simulink model "forty_gbe"  (R2019a)
settings: Solver=VariableStepAuto  StartTime=0.0  StopTime=10.0  RelTol=1e-3
libraries: xbsIndex_r4 x1231, casper_library_misc x9
(part 5 of 14)

== system forty_gbe/forty_gbe/rxs2/arm_delay ==
  d : Inport
  q : Outport
  wires:
  d/1 -> q/1

== system forty_gbe/forty_gbe/rxs2/buscreate ==
  in1 : Inport
  reinterpret1 : xbsIndex_r4/Reinterpret  force_arith_type=on  arith_type=Unsigned  force_bin_pt=on  bin_pt=0  block_type=reinterpret
      settings: infoedit="Changes signal type without altering the binary representation.   You can changed the signal between signed and unsigned, and relocate the binary point.<br><br>Hardware notes: In hardware this block costs nothing.<br><br>Example:  Suppose the input is 6 bits wide, signed, with 2 fractional bits, and the output is forced to unsigned with 0 fractional bits.  Then an input of -2.0 (1110.00 in binary 2's complement) becomes an output of 56 (111000 in binary)."
  bus_out : Outport
  wires:
  in1/1 -> reinterpret1/1
  reinterpret1/1 -> bus_out/1

== system forty_gbe/forty_gbe/rxs2/io_delay ==
  d : Inport
  Register0 : xbsIndex_r4/Register  init=0  rst=off  en=off  dbl_ovrd=off  block_type=register
      settings: block_version=11.4
  Register1 : xbsIndex_r4/Register  init=0  rst=off  en=off  dbl_ovrd=off  block_type=register
      settings: block_version=11.4
  q : Outport
  wires:
  Register1/1 -> q/1
  d/1 -> Register0/1
  Register0/1 -> Register1/1

== system forty_gbe/forty_gbe/rxs2/ss ==
  note: Generate stop
      | when in circular
      | capture mode
  note: Delay start
      | of capture
  note: ctrl:
      | bit0: Put a posedge here
      |         to enable a new capture.
      | bit1: ignore external trigger
      |         and trigger immediately.
      | bit2: ignore external write
      |         enable and capture on
      |         every FPGA clock.
      | bit3: continuously capture
      |         data until we get an
      |         external stop command.
  note: Offset in vector
      | from first element
      | captured, used
      | during circular capture
  note: Number of
      | bytes in
      | buffer and
      | done bit
  note: Number of valid
      | data samples to
      | skip after trigger
      | before starting
      | capture
  note: Value on vin
      | aligned with
      | first sample on
      | din captured
  din : Inport
  we : Inport  Port=2
  trig : Inport  Port=3
  arm : Inport  Port=4
  add_del : xbsIndex_r4/Delay  rst=off  infoeditControl=Selection of Reset will increase slice count due to use of real FFs and instead of SRLs  en=off  latency=1  reg_retiming=on  dbl_ovrd=off  block_type=delay
      settings: block_version=11.4
  add_gen : Subsystem  AncestorBlock=casper_library_scopes/snapshot/add_gen  mask{counter_size=10+4+1, increment=16, nsamples=10, burst_size=0, use_dsp48=on}
      mask prompts: counter_size "Address counter size (2^?)"; increment "Address counter increment"; nsamples "Number of samples (2^?)"; burst_size "Burst size (2^?)"; use_dsp48 "dsp48 counter/s"
      mask init:
      | set_param(gcb,'LinkStatus','inactive');
      | if strcmp(use_dsp48,'on'),
      |     set_param([gcb,'/add_gen'],'implementation','DSP48');
      | else
      |     set_param([gcb,'/add_gen'],'implementation','Fabric');
      | end
  arm_or : xbsIndex_r4/Logical  logical_function=OR  inputs=2  en=off  latency=0  precision=Full  arith_type=Unsigned  n_bits=16  bin_pt=0  align_bp=on  dbl_ovrd=off  block_type=logical
  basic_ctrl : Subsystem  AncestorBlock=casper_library_scopes/snapshot/basic_ctrl  mask{dram=off, data_width=128}
      mask prompts: data_width "data width"
      mask init:
      | set_param(gcb,'LinkStatus','inactive');
      | set_param([gcb,'/dram_munge'], 'dram', dram);
  bram : Subsystem  Tag=xps:bram  AncestorBlock=xps_library/Memory/shared_bram  mask{arith_type=Unsigned, addr_width=10, data_width=128, reg_prim_output=off, reg_core_output=off, optimization=Minimum_Area, data_bin_pt=0, init_vals=[0:2^10-1], sample_rate=1}
      mask prompts: arith_type "Output Data Type"; addr_width "Address width"; data_width "Data Width"; reg_prim_output "Register Primitive Output"; reg_core_output "Register Core Output"; data_bin_pt "Data Binary Point"; init_vals "Initial values (simulation only)"; sample_rate "Sample rate"
      mask init:
      | shared_bram_mask;
      mask TypeOptions arith_type: Unsigned | Signed  (2's comp)
      mask TypeOptions data_width: 8 | 16 | 32 | 64 | 128
      mask TypeOptions optimization: Minimum_Area | Low_Power
  cast : xbsIndex_r4/Convert  gui_display_data_type=Fixed-point  arith_type=Unsigned  n_bits=128  bin_pt=0  float_type=Single  exp_bits=8  fraction_bits=24  quantization=Truncate  overflow=Wrap  en=off  latency=0  pipeline=off  dbl_ovrd=off  block_type=convert
      settings: block_version=11.4
  circ : xbsIndex_r4/Constant  const=0  gui_display_data_type=Fixed-point  arith_type=Boolean  n_bits=16  bin_pt=14  preci_type=Single  exp_width=8  frac_width=24  explicit_period=on  period=1  equ=P=C  opselect=C  inp2=PCIN>>17  opr=+  inp1=P  carry=CIN  dbl_ovrd=off  block_type=constant
  circ_or : xbsIndex_r4/Logical  logical_function=OR  inputs=2  en=off  latency=0  precision=Full  arith_type=Unsigned  n_bits=16  bin_pt=0  align_bp=on  dbl_ovrd=off  block_type=logical
  ctrl : Subsystem  Tag=xps:sw_reg  AncestorBlock=xps_library/Memory/software_register  mask(swreg){io_dir=From Processor, io_delay=0, init_val=0, sample_period=1, names=reg, bitwidths=32, bin_pts=0, arith_types=0, sim_port=off, show_format=on}
      mask prompts: io_dir "I/O direction"; io_delay "I/O delay"; init_val "Initial Value"; sample_period "Sample period"; names "Bitfield names [msb...lsb]"; bitwidths "Bitfield widths"; bin_pts "Bitfield binary pts"; arith_types "Bitfield types, ufix=0, fix=1, bool=2"; sim_port "Provide sim input/output?"; show_format "Print format string?"
      mask help: A 32-bit software-accessible register. Can be divided into bitfields of varying widths and types using the fields in the block mask.
      mask init:
      | swreg_init(gcb)
      settings: AttributesFormatString=1input:uf32.0 = 32 bits
      mask TypeOptions io_dir: To Processor | From Processor
      mask Callback io_dir:
      | mask_enables = get_param(gcb, 'MaskEnables');
      | mask_names = get_param(gcb, 'MaskNames');
      | if strcmp(get_param(gcb, 'io_dir'), 'To Processor'),
      |     mask_enables{ismember(mask_names, 'sample_period')} = 'off';
      | else
      |     mask_enables{ismember(mask_names, 'sample_period')} = 'on';
      | end
      | set_param(gcb, 'MaskEnables', mask_enables);
      mask DialogControl ParameterTabVar0 Prompt: Setup
  ctrl_combine : Subsystem  AncestorBlock=casper_library_flow_control/bus_create  mask(bus_create){inputNum=4}
      mask prompts: inputNum "Number of inputs:"
      mask init:
      | bus_create_init(gcb,...
      |     'inputNum', inputNum);
  ctrl_split : Subsystem  AncestorBlock=casper_library_flow_control/bus_expand  mask(bus_expand){mode=divisions of arbitrary size, outputNum=1, outputWidth=[28 1 2 1], outputBinaryPt=0, outputArithmeticType=[0 2 0 2], show_format=on, outputToWorkspace=off, variablePrefix=out, outputToModelAsWell=on}
      mask prompts: outputNum "Number of outputs:"; outputWidth "Output width [msb ... lsb]:"; outputBinaryPt "Output binary point position [msb ... lsb]:"; outputArithmeticType "Output arithmetic type (ufix=0, fix=1, bool=2) [msb ... lsb]:"; show_format "Print format string?"; outputToWorkspace "Output to workspace?"; variablePrefix "Variable name prefix:"; outputToModelAsWell "Output to model as well?"
      mask help:
      | Expands a 'bus' made using a bus_create or Xilinx
      | concat block.
      | The input will be divided into the specified number
      | of outputs with the specified arithmetic types.
      | Divisions are made from most significant bit.
      mask init: same as forty_gbe/forty_gbe/rx_dv_or_exp
      settings: AttributesFormatString=4 outputs: uf28.0,b,uf2.0,b,
      mask TypeOptions mode: divisions of equal size | divisions of arbitrary size
      mask Callback mode: bus_expand_callback();
      mask Callback outputWidth: bus_expand_callback();
      mask Callback outputToWorkspace: bus_expand_callback();
  dat_del : xbsIndex_r4/Delay  rst=off  infoeditControl=Selection of Reset will increase slice count due to use of real FFs and instead of SRLs  en=off  latency=1  reg_retiming=on  dbl_ovrd=off  block_type=delay
      settings: block_version=11.4
  g_tr_en_cnt : Terminator
  gbram : Terminator
  goto_ss_we2_const : xbsIndex_r4/Constant  const=0  gui_display_data_type=Fixed-point  arith_type=Boolean  n_bits=16  bin_pt=14  preci_type=Single  exp_width=8  frac_width=24  explicit_period=on  period=1  equ=P=C  opselect=C  inp2=PCIN>>17  opr=+  inp1=P  carry=CIN  dbl_ovrd=off  block_type=constant
  goto_ss_we3_const : xbsIndex_r4/Constant  const=0  gui_display_data_type=Fixed-point  arith_type=Boolean  n_bits=16  bin_pt=14  preci_type=Single  exp_width=8  frac_width=24  explicit_period=on  period=1  equ=P=C  opselect=C  inp2=PCIN>>17  opr=+  inp1=P  carry=CIN  dbl_ovrd=off  block_type=constant
  gval : Terminator
  never : xbsIndex_r4/Constant  const=0  gui_display_data_type=Fixed-point  arith_type=Boolean  n_bits=16  bin_pt=14  preci_type=Single  exp_width=8  frac_width=24  explicit_period=on  period=1  equ=P=C  opselect=C  inp2=PCIN>>17  opr=+  inp1=P  carry=CIN  dbl_ovrd=off  block_type=constant
  ri : xbsIndex_r4/Reinterpret  force_arith_type=on  arith_type=Unsigned  force_bin_pt=on  bin_pt=0  block_type=reinterpret
      settings: infoedit="Changes signal type without altering the binary representation.   You can changed the signal between signed and unsigned, and relocate the binary point.<br><br>Hardware notes: In hardware this block costs nothing.<br><br>Example:  Suppose the input is 6 bits wide, signed, with 2 fractional bits, and the output is forced to unsigned with 0 fractional bits.  Then an input of -2.0 (1110.00 in binary 2's complement) becomes an output of 56 (111000 in binary)."
  status : Subsystem  Tag=xps:sw_reg  AncestorBlock=xps_library/Memory/software_register  mask(swreg){io_dir=To Processor, io_delay=0, init_val=0, sample_period=1, names=reg, bitwidths=32, bin_pts=0, arith_types=0, sim_port=off, show_format=on}
      mask prompts: io_dir "I/O direction"; io_delay "I/O delay"; init_val "Initial Value"; sample_period "Sample period"; names "Bitfield names [msb...lsb]"; bitwidths "Bitfield widths"; bin_pts "Bitfield binary pts"; arith_types "Bitfield types, ufix=0, fix=1, bool=2"; sim_port "Provide sim input/output?"; show_format "Print format string?"
      mask help: A 32-bit software-accessible register. Can be divided into bitfields of varying widths and types using the fields in the block mask.
      mask init:
      | swreg_init(gcb)
      settings: AttributesFormatString=1output:uf32.0 = 32 bits
      mask TypeOptions io_dir: To Processor | From Processor
      mask Callback io_dir:
      | mask_enables = get_param(gcb, 'MaskEnables');
      | mask_names = get_param(gcb, 'MaskNames');
      | if strcmp(get_param(gcb, 'io_dir'), 'To Processor'),
      |     mask_enables{ismember(mask_names, 'sample_period')} = 'off';
      | else
      |     mask_enables{ismember(mask_names, 'sample_period')} = 'on';
      | end
      | set_param(gcb, 'MaskEnables', mask_enables);
      mask DialogControl ParameterTabVar0 Prompt: Setup
  vin_const : xbsIndex_r4/Constant  const=0  gui_display_data_type=Fixed-point  arith_type=Boolean  n_bits=16  bin_pt=14  preci_type=Single  exp_width=8  frac_width=24  explicit_period=on  period=1  equ=P=C  opselect=C  inp2=PCIN>>17  opr=+  inp1=P  carry=CIN  dbl_ovrd=off  block_type=constant
  we_del : xbsIndex_r4/Delay  rst=off  infoeditControl=Selection of Reset will increase slice count due to use of real FFs and instead of SRLs  en=off  latency=1  reg_retiming=on  dbl_ovrd=off  block_type=delay
      settings: block_version=11.4
  arm_out : Outport
  tag scope: goto_51569036_we1=global, goto_51569036_we2=global, goto_51569036_we3=global, goto_51569036_we4=global
  wires:
  din/1 -> ri/1
  ri/1 -> cast/1
  cast/1 -> basic_ctrl/2(din)
  we/1 -> basic_ctrl/3(we)
  trig/1 -> basic_ctrl/4(trig)
  ctrl_combine/1(bus_out) -> basic_ctrl/5(ctrl)
  never/1 -> basic_ctrl/6(stopi)
  arm/1 -> arm_or/2
  arm_or/1 -> arm_out/1, ctrl_combine/4(in4)
  circ/1 -> circ_or/2
  ctrl/1(in_reg) -> ctrl_split/1(bus_in)
  ctrl_split/1(msb_out4) -> ctrl_combine/1(in1)
  ctrl_split/2(out3) -> circ_or/1
  ctrl_split/3(out2) -> ctrl_combine/3(in3)
  ctrl_split/4(lsb_out1) -> arm_or/1
  circ_or/1 -> ctrl_combine/2(in2)
  basic_ctrl/1(vout) -> add_gen/1(vin)
  basic_ctrl/2(dout) -> add_gen/2(din)
  basic_ctrl/3(we_o) -> add_gen/3(we), [goto_51569036_we1]
  basic_ctrl/4(go) -> add_gen/4(go)
  basic_ctrl/5(stop) -> add_gen/5(cont)
  basic_ctrl/6(init) -> add_gen/6(init)
  add_gen/5(status) -> status/1(out_reg)
  vin_const/1 -> basic_ctrl/1(vin)
  add_gen/1(vout) -> gval/1
  add_gen/6(en_cnt) -> g_tr_en_cnt/1
  add_gen/2(add) -> add_del/1
  add_gen/3(dout) -> dat_del/1
  add_gen/4(we_o) -> we_del/1, [goto_51569036_we4]
  add_del/1 -> bram/1(addr)
  dat_del/1 -> bram/2(data_in)
  we_del/1 -> bram/3(we)
  bram/1(data_out) -> gbram/1
  goto_ss_we2_const/1 -> [goto_51569036_we2]
  goto_ss_we3_const/1 -> [goto_51569036_we3]

== system forty_gbe/forty_gbe/rxs2/trig_delay ==
  d : Inport
  Register0 : xbsIndex_r4/Register  init=0  rst=off  en=off  dbl_ovrd=off  block_type=register
      settings: block_version=11.4
  Register1 : xbsIndex_r4/Register  init=0  rst=off  en=off  dbl_ovrd=off  block_type=register
      settings: block_version=11.4
  q : Outport
  wires:
  Register1/1 -> q/1
  d/1 -> Register0/1
  Register0/1 -> Register1/1

== system forty_gbe/forty_gbe/rxs2/we_delay ==
  d : Inport
  Register0 : xbsIndex_r4/Register  init=0  rst=off  en=off  dbl_ovrd=off  block_type=register
      settings: block_version=11.4
  Register1 : xbsIndex_r4/Register  init=0  rst=off  en=off  dbl_ovrd=off  block_type=register
      settings: block_version=11.4
  q : Outport
  wires:
  Register1/1 -> q/1
  d/1 -> Register0/1
  Register0/1 -> Register1/1

== system forty_gbe/forty_gbe/rxs3/arm_delay ==
  d : Inport
  q : Outport
  wires:
  d/1 -> q/1

== system forty_gbe/forty_gbe/rxs3/buscreate ==
  in1 : Inport
  in2 : Inport  Port=2
  concatenate : xbsIndex_r4/Concat  num_inputs=2  dbl_ovrd=off  block_type=concat
  reinterpret1 : xbsIndex_r4/Reinterpret  force_arith_type=on  arith_type=Unsigned  force_bin_pt=on  bin_pt=0  block_type=reinterpret
      settings: infoedit="Changes signal type without altering the binary representation.   You can changed the signal between signed and unsigned, and relocate the binary point.<br><br>Hardware notes: In hardware this block costs nothing.<br><br>Example:  Suppose the input is 6 bits wide, signed, with 2 fractional bits, and the output is forced to unsigned with 0 fractional bits.  Then an input of -2.0 (1110.00 in binary 2's complement) becomes an output of 56 (111000 in binary)."
  reinterpret2 : xbsIndex_r4/Reinterpret  force_arith_type=on  arith_type=Unsigned  force_bin_pt=on  bin_pt=0  block_type=reinterpret
      settings: infoedit="Changes signal type without altering the binary representation.   You can changed the signal between signed and unsigned, and relocate the binary point.<br><br>Hardware notes: In hardware this block costs nothing.<br><br>Example:  Suppose the input is 6 bits wide, signed, with 2 fractional bits, and the output is forced to unsigned with 0 fractional bits.  Then an input of -2.0 (1110.00 in binary 2's complement) becomes an output of 56 (111000 in binary)."
  bus_out : Outport
  wires:
  concatenate/1 -> bus_out/1
  in1/1 -> reinterpret1/1
  reinterpret1/1 -> concatenate/1
  in2/1 -> reinterpret2/1
  reinterpret2/1 -> concatenate/2

== system forty_gbe/forty_gbe/rxs3/io_delay ==
  d : Inport
  Register0 : xbsIndex_r4/Register  init=0  rst=off  en=off  dbl_ovrd=off  block_type=register
      settings: block_version=11.4
  Register1 : xbsIndex_r4/Register  init=0  rst=off  en=off  dbl_ovrd=off  block_type=register
      settings: block_version=11.4
  q : Outport
  wires:
  Register1/1 -> q/1
  d/1 -> Register0/1
  Register0/1 -> Register1/1

== system forty_gbe/forty_gbe/rxs3/ss ==
  note: Generate stop
      | when in circular
      | capture mode
  note: Delay start
      | of capture
  note: ctrl:
      | bit0: Put a posedge here
      |         to enable a new capture.
      | bit1: ignore external trigger
      |         and trigger immediately.
      | bit2: ignore external write
      |         enable and capture on
      |         every FPGA clock.
      | bit3: continuously capture
      |         data until we get an
      |         external stop command.
  note: Offset in vector
      | from first element
      | captured, used
      | during circular capture
  note: Number of
      | bytes in
      | buffer and
      | done bit
  note: Number of valid
      | data samples to
      | skip after trigger
      | before starting
      | capture
  note: Value on vin
      | aligned with
      | first sample on
      | din captured
  din : Inport
  we : Inport  Port=2
  trig : Inport  Port=3
  arm : Inport  Port=4
  add_del : xbsIndex_r4/Delay  rst=off  infoeditControl=Selection of Reset will increase slice count due to use of real FFs and instead of SRLs  en=off  latency=1  reg_retiming=on  dbl_ovrd=off  block_type=delay
      settings: block_version=11.4
  add_gen : Subsystem  AncestorBlock=casper_library_scopes/snapshot/add_gen  mask{counter_size=10+3+1, increment=8, nsamples=10, burst_size=0, use_dsp48=on}
      mask prompts: counter_size "Address counter size (2^?)"; increment "Address counter increment"; nsamples "Number of samples (2^?)"; burst_size "Burst size (2^?)"; use_dsp48 "dsp48 counter/s"
      mask init:
      | set_param(gcb,'LinkStatus','inactive');
      | if strcmp(use_dsp48,'on'),
      |     set_param([gcb,'/add_gen'],'implementation','DSP48');
      | else
      |     set_param([gcb,'/add_gen'],'implementation','Fabric');
      | end
  arm_or : xbsIndex_r4/Logical  logical_function=OR  inputs=2  en=off  latency=0  precision=Full  arith_type=Unsigned  n_bits=16  bin_pt=0  align_bp=on  dbl_ovrd=off  block_type=logical
  basic_ctrl : Subsystem  AncestorBlock=casper_library_scopes/snapshot/basic_ctrl  mask{dram=off, data_width=64}
      mask prompts: data_width "data width"
      mask init:
      | set_param(gcb,'LinkStatus','inactive');
      | set_param([gcb,'/dram_munge'], 'dram', dram);
  bram : Subsystem  Tag=xps:bram  AncestorBlock=xps_library/Memory/shared_bram  mask{arith_type=Unsigned, addr_width=10, data_width=64, reg_prim_output=off, reg_core_output=off, optimization=Minimum_Area, data_bin_pt=0, init_vals=[0:2^10-1], sample_rate=1}
      mask prompts: arith_type "Output Data Type"; addr_width "Address width"; data_width "Data Width"; reg_prim_output "Register Primitive Output"; reg_core_output "Register Core Output"; data_bin_pt "Data Binary Point"; init_vals "Initial values (simulation only)"; sample_rate "Sample rate"
      mask init:
      | shared_bram_mask;
      mask TypeOptions arith_type: Unsigned | Signed  (2's comp)
      mask TypeOptions data_width: 8 | 16 | 32 | 64 | 128
      mask TypeOptions optimization: Minimum_Area | Low_Power
  cast : xbsIndex_r4/Convert  gui_display_data_type=Fixed-point  arith_type=Unsigned  n_bits=64  bin_pt=0  float_type=Single  exp_bits=8  fraction_bits=24  quantization=Truncate  overflow=Wrap  en=off  latency=0  pipeline=off  dbl_ovrd=off  block_type=convert
      settings: block_version=11.4
  circ : xbsIndex_r4/Constant  const=0  gui_display_data_type=Fixed-point  arith_type=Boolean  n_bits=16  bin_pt=14  preci_type=Single  exp_width=8  frac_width=24  explicit_period=on  period=1  equ=P=C  opselect=C  inp2=PCIN>>17  opr=+  inp1=P  carry=CIN  dbl_ovrd=off  block_type=constant
  circ_or : xbsIndex_r4/Logical  logical_function=OR  inputs=2  en=off  latency=0  precision=Full  arith_type=Unsigned  n_bits=16  bin_pt=0  align_bp=on  dbl_ovrd=off  block_type=logical
  ctrl : Subsystem  Tag=xps:sw_reg  AncestorBlock=xps_library/Memory/software_register  mask(swreg){io_dir=From Processor, io_delay=0, init_val=0, sample_period=1, names=reg, bitwidths=32, bin_pts=0, arith_types=0, sim_port=off, show_format=on}
      mask prompts: io_dir "I/O direction"; io_delay "I/O delay"; init_val "Initial Value"; sample_period "Sample period"; names "Bitfield names [msb...lsb]"; bitwidths "Bitfield widths"; bin_pts "Bitfield binary pts"; arith_types "Bitfield types, ufix=0, fix=1, bool=2"; sim_port "Provide sim input/output?"; show_format "Print format string?"
      mask help: A 32-bit software-accessible register. Can be divided into bitfields of varying widths and types using the fields in the block mask.
      mask init:
      | swreg_init(gcb)
      settings: AttributesFormatString=1input:uf32.0 = 32 bits
      mask TypeOptions io_dir: To Processor | From Processor
      mask Callback io_dir:
      | mask_enables = get_param(gcb, 'MaskEnables');
      | mask_names = get_param(gcb, 'MaskNames');
      | if strcmp(get_param(gcb, 'io_dir'), 'To Processor'),
      |     mask_enables{ismember(mask_names, 'sample_period')} = 'off';
      | else
      |     mask_enables{ismember(mask_names, 'sample_period')} = 'on';
      | end
      | set_param(gcb, 'MaskEnables', mask_enables);
      mask DialogControl ParameterTabVar0 Prompt: Setup
  ctrl_combine : Subsystem  AncestorBlock=casper_library_flow_control/bus_create  mask(bus_create){inputNum=4}
      mask prompts: inputNum "Number of inputs:"
      mask init:
      | bus_create_init(gcb,...
      |     'inputNum', inputNum);
  ctrl_split : Subsystem  AncestorBlock=casper_library_flow_control/bus_expand  mask(bus_expand){mode=divisions of arbitrary size, outputNum=1, outputWidth=[28 1 2 1], outputBinaryPt=0, outputArithmeticType=[0 2 0 2], show_format=on, outputToWorkspace=off, variablePrefix=out, outputToModelAsWell=on}
      mask prompts: outputNum "Number of outputs:"; outputWidth "Output width [msb ... lsb]:"; outputBinaryPt "Output binary point position [msb ... lsb]:"; outputArithmeticType "Output arithmetic type (ufix=0, fix=1, bool=2) [msb ... lsb]:"; show_format "Print format string?"; outputToWorkspace "Output to workspace?"; variablePrefix "Variable name prefix:"; outputToModelAsWell "Output to model as well?"
      mask help:
      | Expands a 'bus' made using a bus_create or Xilinx
      | concat block.
      | The input will be divided into the specified number
      | of outputs with the specified arithmetic types.
      | Divisions are made from most significant bit.
      mask init: same as forty_gbe/forty_gbe/rx_dv_or_exp
      settings: AttributesFormatString=4 outputs: uf28.0,b,uf2.0,b,
      mask TypeOptions mode: divisions of equal size | divisions of arbitrary size
      mask Callback mode: bus_expand_callback();
      mask Callback outputWidth: bus_expand_callback();
      mask Callback outputToWorkspace: bus_expand_callback();
  dat_del : xbsIndex_r4/Delay  rst=off  infoeditControl=Selection of Reset will increase slice count due to use of real FFs and instead of SRLs  en=off  latency=1  reg_retiming=on  dbl_ovrd=off  block_type=delay
      settings: block_version=11.4
  g_tr_en_cnt : Terminator
  gbram : Terminator
  goto_ss_we2_const : xbsIndex_r4/Constant  const=0  gui_display_data_type=Fixed-point  arith_type=Boolean  n_bits=16  bin_pt=14  preci_type=Single  exp_width=8  frac_width=24  explicit_period=on  period=1  equ=P=C  opselect=C  inp2=PCIN>>17  opr=+  inp1=P  carry=CIN  dbl_ovrd=off  block_type=constant
  goto_ss_we3_const : xbsIndex_r4/Constant  const=0  gui_display_data_type=Fixed-point  arith_type=Boolean  n_bits=16  bin_pt=14  preci_type=Single  exp_width=8  frac_width=24  explicit_period=on  period=1  equ=P=C  opselect=C  inp2=PCIN>>17  opr=+  inp1=P  carry=CIN  dbl_ovrd=off  block_type=constant
  gval : Terminator
  never : xbsIndex_r4/Constant  const=0  gui_display_data_type=Fixed-point  arith_type=Boolean  n_bits=16  bin_pt=14  preci_type=Single  exp_width=8  frac_width=24  explicit_period=on  period=1  equ=P=C  opselect=C  inp2=PCIN>>17  opr=+  inp1=P  carry=CIN  dbl_ovrd=off  block_type=constant
  ri : xbsIndex_r4/Reinterpret  force_arith_type=on  arith_type=Unsigned  force_bin_pt=on  bin_pt=0  block_type=reinterpret
      settings: infoedit="Changes signal type without altering the binary representation.   You can changed the signal between signed and unsigned, and relocate the binary point.<br><br>Hardware notes: In hardware this block costs nothing.<br><br>Example:  Suppose the input is 6 bits wide, signed, with 2 fractional bits, and the output is forced to unsigned with 0 fractional bits.  Then an input of -2.0 (1110.00 in binary 2's complement) becomes an output of 56 (111000 in binary)."
  status : Subsystem  Tag=xps:sw_reg  AncestorBlock=xps_library/Memory/software_register  mask(swreg){io_dir=To Processor, io_delay=0, init_val=0, sample_period=1, names=reg, bitwidths=32, bin_pts=0, arith_types=0, sim_port=off, show_format=on}
      mask prompts: io_dir "I/O direction"; io_delay "I/O delay"; init_val "Initial Value"; sample_period "Sample period"; names "Bitfield names [msb...lsb]"; bitwidths "Bitfield widths"; bin_pts "Bitfield binary pts"; arith_types "Bitfield types, ufix=0, fix=1, bool=2"; sim_port "Provide sim input/output?"; show_format "Print format string?"
      mask help: A 32-bit software-accessible register. Can be divided into bitfields of varying widths and types using the fields in the block mask.
      mask init:
      | swreg_init(gcb)
      settings: AttributesFormatString=1output:uf32.0 = 32 bits
      mask TypeOptions io_dir: To Processor | From Processor
      mask Callback io_dir:
      | mask_enables = get_param(gcb, 'MaskEnables');
      | mask_names = get_param(gcb, 'MaskNames');
      | if strcmp(get_param(gcb, 'io_dir'), 'To Processor'),
      |     mask_enables{ismember(mask_names, 'sample_period')} = 'off';
      | else
      |     mask_enables{ismember(mask_names, 'sample_period')} = 'on';
      | end
      | set_param(gcb, 'MaskEnables', mask_enables);
      mask DialogControl ParameterTabVar0 Prompt: Setup
  vin_const : xbsIndex_r4/Constant  const=0  gui_display_data_type=Fixed-point  arith_type=Boolean  n_bits=16  bin_pt=14  preci_type=Single  exp_width=8  frac_width=24  explicit_period=on  period=1  equ=P=C  opselect=C  inp2=PCIN>>17  opr=+  inp1=P  carry=CIN  dbl_ovrd=off  block_type=constant
  we_del : xbsIndex_r4/Delay  rst=off  infoeditControl=Selection of Reset will increase slice count due to use of real FFs and instead of SRLs  en=off  latency=1  reg_retiming=on  dbl_ovrd=off  block_type=delay
      settings: block_version=11.4
  arm_out : Outport
  tag scope: goto_51598827_we1=global, goto_51598827_we2=global, goto_51598827_we3=global, goto_51598827_we4=global
  wires:
  din/1 -> ri/1
  ri/1 -> cast/1
  cast/1 -> basic_ctrl/2(din)
  we/1 -> basic_ctrl/3(we)
  trig/1 -> basic_ctrl/4(trig)
  ctrl_combine/1(bus_out) -> basic_ctrl/5(ctrl)
  never/1 -> basic_ctrl/6(stopi)
  arm/1 -> arm_or/2
  arm_or/1 -> arm_out/1, ctrl_combine/4(in4)
  circ/1 -> circ_or/2
  ctrl/1(in_reg) -> ctrl_split/1(bus_in)
  ctrl_split/1(msb_out4) -> ctrl_combine/1(in1)
  ctrl_split/2(out3) -> circ_or/1
  ctrl_split/3(out2) -> ctrl_combine/3(in3)
  ctrl_split/4(lsb_out1) -> arm_or/1
  circ_or/1 -> ctrl_combine/2(in2)
  basic_ctrl/1(vout) -> add_gen/1(vin)
  basic_ctrl/2(dout) -> add_gen/2(din)
  basic_ctrl/3(we_o) -> add_gen/3(we), [goto_51598827_we1]
  basic_ctrl/4(go) -> add_gen/4(go)
  basic_ctrl/5(stop) -> add_gen/5(cont)
  basic_ctrl/6(init) -> add_gen/6(init)
  add_gen/5(status) -> status/1(out_reg)
  vin_const/1 -> basic_ctrl/1(vin)
  add_gen/1(vout) -> gval/1
  add_gen/6(en_cnt) -> g_tr_en_cnt/1
  add_gen/2(add) -> add_del/1
  add_gen/3(dout) -> dat_del/1
  add_gen/4(we_o) -> we_del/1, [goto_51598827_we4]
  add_del/1 -> bram/1(addr)
  dat_del/1 -> bram/2(data_in)
  we_del/1 -> bram/3(we)
  bram/1(data_out) -> gbram/1
  goto_ss_we2_const/1 -> [goto_51598827_we2]
  goto_ss_we3_const/1 -> [goto_51598827_we3]

== system forty_gbe/forty_gbe/rxs3/trig_delay ==
  d : Inport
  Register0 : xbsIndex_r4/Register  init=0  rst=off  en=off  dbl_ovrd=off  block_type=register
      settings: block_version=11.4
  Register1 : xbsIndex_r4/Register  init=0  rst=off  en=off  dbl_ovrd=off  block_type=register
      settings: block_version=11.4
  q : Outport
  wires:
  Register1/1 -> q/1
  d/1 -> Register0/1
  Register0/1 -> Register1/1

== system forty_gbe/forty_gbe/rxs3/we_delay ==
  d : Inport
  Register0 : xbsIndex_r4/Register  init=0  rst=off  en=off  dbl_ovrd=off  block_type=register
      settings: block_version=11.4
  Register1 : xbsIndex_r4/Register  init=0  rst=off  en=off  dbl_ovrd=off  block_type=register
      settings: block_version=11.4
  q : Outport
  wires:
  Register1/1 -> q/1
  d/1 -> Register0/1
  Register0/1 -> Register1/1

== system forty_gbe/forty_gbe/txs0/buscreate ==
  in1 : Inport
  in2 : Inport  Port=2
  in3 : Inport  Port=3
  in4 : Inport  Port=4
  in5 : Inport  Port=5
  in6 : Inport  Port=6
  in7 : Inport  Port=7
  concatenate : xbsIndex_r4/Concat  num_inputs=7  dbl_ovrd=off  block_type=concat
  reinterpret{1..7} (7 alike) : xbsIndex_r4/Reinterpret  force_arith_type=on  arith_type=Unsigned  force_bin_pt=on  bin_pt=0  block_type=reinterpret
      reinterpret1 settings: infoedit="Changes signal type without altering the binary representation.   You can changed the signal between signed and unsigned, and relocate the binary point.<br><br>Hardware notes: In hardware this block costs nothing.<br><br>Example:  Suppose the input is 6 bits wide, signed, with 2 fractional bits, and the output is forced to unsigned with 0 fractional bits.  Then an input of -2.0 (1110.00 in binary 2's complement) becomes an output of 56 (111000 in binary)."
      reinterpret2 settings: infoedit="Changes signal type without altering the binary representation.   You can changed the signal between signed and unsigned, and relocate the binary point.<br><br>Hardware notes: In hardware this block costs nothing.<br><br>Example:  Suppose the input is 6 bits wide, signed, with 2 fractional bits, and the output is forced to unsigned with 0 fractional bits.  Then an input of -2.0 (1110.00 in binary 2's complement) becomes an output of 56 (111000 in binary)."
  bus_out : Outport
  wires:
  concatenate/1 -> bus_out/1
  in1/1 -> reinterpret1/1
  reinterpret1/1 -> concatenate/1
  in2/1 -> reinterpret2/1
  reinterpret2/1 -> concatenate/2
  in3/1 -> reinterpret3/1
  reinterpret3/1 -> concatenate/3
  in4/1 -> reinterpret4/1
  reinterpret4/1 -> concatenate/4
  in5/1 -> reinterpret5/1
  reinterpret5/1 -> concatenate/5
  in6/1 -> reinterpret6/1
  reinterpret6/1 -> concatenate/6
  in7/1 -> reinterpret7/1
  reinterpret7/1 -> concatenate/7

== system forty_gbe/forty_gbe/txs0/io_delay ==
  d : Inport
  Register0 : xbsIndex_r4/Register  init=0  rst=off  en=off  dbl_ovrd=off  block_type=register
      settings: block_version=11.4
  Register1 : xbsIndex_r4/Register  init=0  rst=off  en=off  dbl_ovrd=off  block_type=register
      settings: block_version=11.4
  q : Outport
  wires:
  Register1/1 -> q/1
  d/1 -> Register0/1
  Register0/1 -> Register1/1

== system forty_gbe/forty_gbe/txs0/ss ==
  note: Generate stop
      | when in circular
      | capture mode
  note: Delay start
      | of capture
  note: ctrl:
      | bit0: Put a posedge here
      |         to enable a new capture.
      | bit1: ignore external trigger
      |         and trigger immediately.
      | bit2: ignore external write
      |         enable and capture on
      |         every FPGA clock.
      | bit3: continuously capture
      |         data until we get an
      |         external stop command.
  note: Offset in vector
      | from first element
      | captured, used
      | during circular capture
  note: Number of
      | bytes in
      | buffer and
      | done bit
  note: Number of valid
      | data samples to
      | skip after trigger
      | before starting
      | capture
  note: Value on vin
      | aligned with
      | first sample on
      | din captured
  din : Inport
  we : Inport  Port=2
  trig : Inport  Port=3
  add_del : xbsIndex_r4/Delay  rst=off  infoeditControl=Selection of Reset will increase slice count due to use of real FFs and instead of SRLs  en=off  latency=1  reg_retiming=on  dbl_ovrd=off  block_type=delay
      settings: block_version=11.4
  add_gen : Subsystem  AncestorBlock=casper_library_scopes/snapshot/add_gen  mask{counter_size=10+3+1, increment=8, nsamples=10, burst_size=0, use_dsp48=on}
      mask prompts: counter_size "Address counter size (2^?)"; increment "Address counter increment"; nsamples "Number of samples (2^?)"; burst_size "Burst size (2^?)"; use_dsp48 "dsp48 counter/s"
      mask init:
      | set_param(gcb,'LinkStatus','inactive');
      | if strcmp(use_dsp48,'on'),
      |     set_param([gcb,'/add_gen'],'implementation','DSP48');
      | else
      |     set_param([gcb,'/add_gen'],'implementation','Fabric');
      | end
  arm : xbsIndex_r4/Constant  const=0  gui_display_data_type=Fixed-point  arith_type=Boolean  n_bits=16  bin_pt=14  preci_type=Single  exp_width=8  frac_width=24  explicit_period=on  period=1  equ=P=C  opselect=C  inp2=PCIN>>17  opr=+  inp1=P  carry=CIN  dbl_ovrd=off  block_type=constant
  arm_or : xbsIndex_r4/Logical  logical_function=OR  inputs=2  en=off  latency=0  precision=Full  arith_type=Unsigned  n_bits=16  bin_pt=0  align_bp=on  dbl_ovrd=off  block_type=logical
  basic_ctrl : Subsystem  AncestorBlock=casper_library_scopes/snapshot/basic_ctrl  mask{dram=off, data_width=64}
      mask prompts: data_width "data width"
      mask init:
      | set_param(gcb,'LinkStatus','inactive');
      | set_param([gcb,'/dram_munge'], 'dram', dram);
  bram : Subsystem  Tag=xps:bram  AncestorBlock=xps_library/Memory/shared_bram  mask{arith_type=Unsigned, addr_width=10, data_width=64, reg_prim_output=off, reg_core_output=off, optimization=Minimum_Area, data_bin_pt=0, init_vals=[0:2^10-1], sample_rate=1}
      mask prompts: arith_type "Output Data Type"; addr_width "Address width"; data_width "Data Width"; reg_prim_output "Register Primitive Output"; reg_core_output "Register Core Output"; data_bin_pt "Data Binary Point"; init_vals "Initial values (simulation only)"; sample_rate "Sample rate"
      mask init:
      | shared_bram_mask;
      mask TypeOptions arith_type: Unsigned | Signed  (2's comp)
      mask TypeOptions data_width: 8 | 16 | 32 | 64 | 128
      mask TypeOptions optimization: Minimum_Area | Low_Power
  cast : xbsIndex_r4/Convert  gui_display_data_type=Fixed-point  arith_type=Unsigned  n_bits=64  bin_pt=0  float_type=Single  exp_bits=8  fraction_bits=24  quantization=Truncate  overflow=Wrap  en=off  latency=0  pipeline=off  dbl_ovrd=off  block_type=convert
      settings: block_version=11.4
  circ : xbsIndex_r4/Constant  const=0  gui_display_data_type=Fixed-point  arith_type=Boolean  n_bits=16  bin_pt=14  preci_type=Single  exp_width=8  frac_width=24  explicit_period=on  period=1  equ=P=C  opselect=C  inp2=PCIN>>17  opr=+  inp1=P  carry=CIN  dbl_ovrd=off  block_type=constant
  circ_or : xbsIndex_r4/Logical  logical_function=OR  inputs=2  en=off  latency=0  precision=Full  arith_type=Unsigned  n_bits=16  bin_pt=0  align_bp=on  dbl_ovrd=off  block_type=logical
  ctrl : Subsystem  Tag=xps:sw_reg  AncestorBlock=xps_library/Memory/software_register  mask(swreg){io_dir=From Processor, io_delay=0, init_val=0, sample_period=1, names=reg, bitwidths=32, bin_pts=0, arith_types=0, sim_port=off, show_format=on}
      mask prompts: io_dir "I/O direction"; io_delay "I/O delay"; init_val "Initial Value"; sample_period "Sample period"; names "Bitfield names [msb...lsb]"; bitwidths "Bitfield widths"; bin_pts "Bitfield binary pts"; arith_types "Bitfield types, ufix=0, fix=1, bool=2"; sim_port "Provide sim input/output?"; show_format "Print format string?"
      mask help: A 32-bit software-accessible register. Can be divided into bitfields of varying widths and types using the fields in the block mask.
      mask init:
      | swreg_init(gcb)
      settings: AttributesFormatString=1input:uf32.0 = 32 bits
      mask TypeOptions io_dir: To Processor | From Processor
      mask Callback io_dir:
      | mask_enables = get_param(gcb, 'MaskEnables');
      | mask_names = get_param(gcb, 'MaskNames');
      | if strcmp(get_param(gcb, 'io_dir'), 'To Processor'),
      |     mask_enables{ismember(mask_names, 'sample_period')} = 'off';
      | else
      |     mask_enables{ismember(mask_names, 'sample_period')} = 'on';
      | end
      | set_param(gcb, 'MaskEnables', mask_enables);
      mask DialogControl ParameterTabVar0 Prompt: Setup
  ctrl_combine : Subsystem  AncestorBlock=casper_library_flow_control/bus_create  mask(bus_create){inputNum=4}
      mask prompts: inputNum "Number of inputs:"
      mask init:
      | bus_create_init(gcb,...
      |     'inputNum', inputNum);
  ctrl_split : Subsystem  AncestorBlock=casper_library_flow_control/bus_expand  mask(bus_expand){mode=divisions of arbitrary size, outputNum=1, outputWidth=[28 1 2 1], outputBinaryPt=0, outputArithmeticType=[0 2 0 2], show_format=on, outputToWorkspace=off, variablePrefix=out, outputToModelAsWell=on}
      mask prompts: outputNum "Number of outputs:"; outputWidth "Output width [msb ... lsb]:"; outputBinaryPt "Output binary point position [msb ... lsb]:"; outputArithmeticType "Output arithmetic type (ufix=0, fix=1, bool=2) [msb ... lsb]:"; show_format "Print format string?"; outputToWorkspace "Output to workspace?"; variablePrefix "Variable name prefix:"; outputToModelAsWell "Output to model as well?"
      mask help:
      | Expands a 'bus' made using a bus_create or Xilinx
      | concat block.
      | The input will be divided into the specified number
      | of outputs with the specified arithmetic types.
      | Divisions are made from most significant bit.
      mask init: same as forty_gbe/forty_gbe/rx_dv_or_exp
      settings: AttributesFormatString=4 outputs: uf28.0,b,uf2.0,b,
      mask TypeOptions mode: divisions of equal size | divisions of arbitrary size
      mask Callback mode: bus_expand_callback();
      mask Callback outputWidth: bus_expand_callback();
      mask Callback outputToWorkspace: bus_expand_callback();
  dat_del : xbsIndex_r4/Delay  rst=off  infoeditControl=Selection of Reset will increase slice count due to use of real FFs and instead of SRLs  en=off  latency=1  reg_retiming=on  dbl_ovrd=off  block_type=delay
      settings: block_version=11.4
  g_tr_en_cnt : Terminator
  gbram : Terminator
  goto_ss_we2_const : xbsIndex_r4/Constant  const=0  gui_display_data_type=Fixed-point  arith_type=Boolean  n_bits=16  bin_pt=14  preci_type=Single  exp_width=8  frac_width=24  explicit_period=on  period=1  equ=P=C  opselect=C  inp2=PCIN>>17  opr=+  inp1=P  carry=CIN  dbl_ovrd=off  block_type=constant
  goto_ss_we3_const : xbsIndex_r4/Constant  const=0  gui_display_data_type=Fixed-point  arith_type=Boolean  n_bits=16  bin_pt=14  preci_type=Single  exp_width=8  frac_width=24  explicit_period=on  period=1  equ=P=C  opselect=C  inp2=PCIN>>17  opr=+  inp1=P  carry=CIN  dbl_ovrd=off  block_type=constant
  gval : Terminator
  never : xbsIndex_r4/Constant  const=0  gui_display_data_type=Fixed-point  arith_type=Boolean  n_bits=16  bin_pt=14  preci_type=Single  exp_width=8  frac_width=24  explicit_period=on  period=1  equ=P=C  opselect=C  inp2=PCIN>>17  opr=+  inp1=P  carry=CIN  dbl_ovrd=off  block_type=constant
  ri : xbsIndex_r4/Reinterpret  force_arith_type=on  arith_type=Unsigned  force_bin_pt=on  bin_pt=0  block_type=reinterpret
      settings: infoedit="Changes signal type without altering the binary representation.   You can changed the signal between signed and unsigned, and relocate the binary point.<br><br>Hardware notes: In hardware this block costs nothing.<br><br>Example:  Suppose the input is 6 bits wide, signed, with 2 fractional bits, and the output is forced to unsigned with 0 fractional bits.  Then an input of -2.0 (1110.00 in binary 2's complement) becomes an output of 56 (111000 in binary)."
  status : Subsystem  Tag=xps:sw_reg  AncestorBlock=xps_library/Memory/software_register  mask(swreg){io_dir=To Processor, io_delay=0, init_val=0, sample_period=1, names=reg, bitwidths=32, bin_pts=0, arith_types=0, sim_port=off, show_format=on}
      mask prompts: io_dir "I/O direction"; io_delay "I/O delay"; init_val "Initial Value"; sample_period "Sample period"; names "Bitfield names [msb...lsb]"; bitwidths "Bitfield widths"; bin_pts "Bitfield binary pts"; arith_types "Bitfield types, ufix=0, fix=1, bool=2"; sim_port "Provide sim input/output?"; show_format "Print format string?"
      mask help: A 32-bit software-accessible register. Can be divided into bitfields of varying widths and types using the fields in the block mask.
      mask init:
      | swreg_init(gcb)
      settings: AttributesFormatString=1output:uf32.0 = 32 bits
      mask TypeOptions io_dir: To Processor | From Processor
      mask Callback io_dir:
      | mask_enables = get_param(gcb, 'MaskEnables');
      | mask_names = get_param(gcb, 'MaskNames');
      | if strcmp(get_param(gcb, 'io_dir'), 'To Processor'),
      |     mask_enables{ismember(mask_names, 'sample_period')} = 'off';
      | else
      |     mask_enables{ismember(mask_names, 'sample_period')} = 'on';
      | end
      | set_param(gcb, 'MaskEnables', mask_enables);
      mask DialogControl ParameterTabVar0 Prompt: Setup
  vin_const : xbsIndex_r4/Constant  const=0  gui_display_data_type=Fixed-point  arith_type=Boolean  n_bits=16  bin_pt=14  preci_type=Single  exp_width=8  frac_width=24  explicit_period=on  period=1  equ=P=C  opselect=C  inp2=PCIN>>17  opr=+  inp1=P  carry=CIN  dbl_ovrd=off  block_type=constant
  we_del : xbsIndex_r4/Delay  rst=off  infoeditControl=Selection of Reset will increase slice count due to use of real FFs and instead of SRLs  en=off  latency=1  reg_retiming=on  dbl_ovrd=off  block_type=delay
      settings: block_version=11.4
  arm_out : Outport
  tag scope: goto_81686352_we1=global, goto_81686352_we2=global, goto_81686352_we3=global, goto_81686352_we4=global
  wires:
  din/1 -> ri/1
  ri/1 -> cast/1
  cast/1 -> basic_ctrl/2(din)
  we/1 -> basic_ctrl/3(we)
  trig/1 -> basic_ctrl/4(trig)
  ctrl_combine/1(bus_out) -> basic_ctrl/5(ctrl)
  never/1 -> basic_ctrl/6(stopi)
  arm/1 -> arm_or/2
  arm_or/1 -> arm_out/1, ctrl_combine/4(in4)
  circ/1 -> circ_or/2
  ctrl/1(in_reg) -> ctrl_split/1(bus_in)
  ctrl_split/1(msb_out4) -> ctrl_combine/1(in1)
  ctrl_split/2(out3) -> circ_or/1
  ctrl_split/3(out2) -> ctrl_combine/3(in3)
  ctrl_split/4(lsb_out1) -> arm_or/1
  circ_or/1 -> ctrl_combine/2(in2)
  basic_ctrl/1(vout) -> add_gen/1(vin)
  basic_ctrl/2(dout) -> add_gen/2(din)
  basic_ctrl/3(we_o) -> add_gen/3(we), [goto_81686352_we1]
  basic_ctrl/4(go) -> add_gen/4(go)
  basic_ctrl/5(stop) -> add_gen/5(cont)
  basic_ctrl/6(init) -> add_gen/6(init)
  add_gen/5(status) -> status/1(out_reg)
  vin_const/1 -> basic_ctrl/1(vin)
  add_gen/1(vout) -> gval/1
  add_gen/6(en_cnt) -> g_tr_en_cnt/1
  add_gen/2(add) -> add_del/1
  add_gen/3(dout) -> dat_del/1
  add_gen/4(we_o) -> we_del/1, [goto_81686352_we4]
  add_del/1 -> bram/1(addr)
  dat_del/1 -> bram/2(data_in)
  we_del/1 -> bram/3(we)
  bram/1(data_out) -> gbram/1
  goto_ss_we2_const/1 -> [goto_81686352_we2]
  goto_ss_we3_const/1 -> [goto_81686352_we3]

== system forty_gbe/forty_gbe/txs0/trig_delay ==
  d : Inport
  Register0 : xbsIndex_r4/Register  init=0  rst=off  en=off  dbl_ovrd=off  block_type=register
      settings: block_version=11.4
  Register1 : xbsIndex_r4/Register  init=0  rst=off  en=off  dbl_ovrd=off  block_type=register
      settings: block_version=11.4
  q : Outport
  wires:
  Register1/1 -> q/1
  d/1 -> Register0/1
  Register0/1 -> Register1/1

== system forty_gbe/forty_gbe/txs0/we_delay ==
  d : Inport
  Register0 : xbsIndex_r4/Register  init=0  rst=off  en=off  dbl_ovrd=off  block_type=register
      settings: block_version=11.4
  Register1 : xbsIndex_r4/Register  init=0  rst=off  en=off  dbl_ovrd=off  block_type=register
      settings: block_version=11.4
  q : Outport
  wires:
  Register1/1 -> q/1
  d/1 -> Register0/1
  Register0/1 -> Register1/1

== system forty_gbe/forty_gbe/txs1/arm_delay ==
  d : Inport
  q : Outport
  wires:
  d/1 -> q/1

== system forty_gbe/forty_gbe/txs1/buscreate ==
  in1 : Inport
  reinterpret1 : xbsIndex_r4/Reinterpret  force_arith_type=on  arith_type=Unsigned  force_bin_pt=on  bin_pt=0  block_type=reinterpret
      settings: infoedit="Changes signal type without altering the binary representation.   You can changed the signal between signed and unsigned, and relocate the binary point.<br><br>Hardware notes: In hardware this block costs nothing.<br><br>Example:  Suppose the input is 6 bits wide, signed, with 2 fractional bits, and the output is forced to unsigned with 0 fractional bits.  Then an input of -2.0 (1110.00 in binary 2's complement) becomes an output of 56 (111000 in binary)."
  bus_out : Outport
  wires:
  in1/1 -> reinterpret1/1
  reinterpret1/1 -> bus_out/1

== system forty_gbe/forty_gbe/txs1/io_delay ==
  d : Inport
  Register0 : xbsIndex_r4/Register  init=0  rst=off  en=off  dbl_ovrd=off  block_type=register
      settings: block_version=11.4
  Register1 : xbsIndex_r4/Register  init=0  rst=off  en=off  dbl_ovrd=off  block_type=register
      settings: block_version=11.4
  q : Outport
  wires:
  Register1/1 -> q/1
  d/1 -> Register0/1
  Register0/1 -> Register1/1
